simulink model "sf_car"  (R2025b)
settings: Solver=ode5  StartTime=0.0  StopTime=100  RelTol=1e-3  AbsTol=1e-6
model workspace (MAT data in the model file):
  Iei = 0.0219914882836
  converter_data = [0  137.465208994  2.232; 0.1  137.065019157  2.075; 0.2  135.864449646  1.975; 0.3  135.664354728  1.846; 0.4  137.565256453  1.72; 0.5  140.366585312  1.564; 0.6  145.268910814  1.409; 0.7  152.872517717  1.254; 0.8  162.9773111  1.096; 0.81  164.27792807  1.08; 0.82  166.178829795  1.061; 0.83  167.979684062  1.043; 0.84  170.080680706  1.028; 0.85  172.781962105  1.012; 0.86  175.383196045  1.002; 0.87  179.585189333  1.002; 0.88  183.587087703  1.001; 0.89  189.890077635  0.998; 0.9  197.693779455  0.999; 0.92  215.902417037  1.001; 0.94  244.515990379  1.002]
  downtab = [0  5  20  35; 0  5  20  35; 0  5  25  40; 0  5  30  50; 0  30  50  80; 0  30  50  80]
  downth = [0; 5; 40; 50; 90; 100]
  emap = [-40  -44  -49  -53  -57  -61  -65  -70  -74  -78  -82; 215  117  85  66  44  29  10  -2  -13  -22  -32; 245  208  178  148  122  104  85  66  48  33  18; 264  260  241  219  193  167  152  133  119  96  85; 264  279  282  275  260  238  223  208  189  171  152; 267  290  293  297  290  275  260  256  234  212  193; 267  297  305  305  305  301  293  282  267  249  226; 267  301  308  312  319  323  319  316  297  279  253; 267  301  312  319  327  327  327  327  312  293  267; 267  301  312  319  327  334  334  334  319  305  275]
  nevec = [800 1200 1600 2000 2400 2800 3200 3600 4000 4400 4800]
  p0 = 0.07934
  p1 = 0.07934
  thvec = [0; 20; 30; 40; 50; 60; 70; 80; 90; 100]
  uptab = [10  30  50  1000000; 10  30  50  1000000; 15  30  50  1000000; 23  41  60  1000000; 40  70  100  1000000; 40  70  100  1000000]
  upth = [0; 25; 35; 50; 90; 100]
  vehicledata = [3.23; 40; 0.3; 1; 50; 0]
libraries: SignalEditorBlockLib x1
settings Model: ExtModeTrigMode=oneshot  ExtModeArmWhenConnect=off  ExtModeAutoUpdateStatusClock=off  Creator=The MathWorks, Inc.  LastModifiedBy=The MathWorks, Inc.
settings SolverCC: AutoScaleAbsTol=off  AlgebraicLoopSolver=TrustRegion
settings DataIOCC: SaveFormat=Array  SaveOutput=off  SaveTime=off  ReturnWorkspaceOutputs=off  SignalLoggingName=sigsOut
settings OptimizationCC: BlockReduction=off  BooleanDataType=off  ExpressionDepthLimit=2147483647.0  InitFltsAndDblsToZero=on  EfficientMapNaN2IntZero=off  LifeSpan=inf
settings DebuggingCC: SaveWithParameterizedLinksMsg=none  UnderspecifiedInitializationDetection=Classic  MergeDetectMultiDrivingBlocksExec=none  CheckExecutionContextPreStartOutputMsg=on  SignalResolutionControl=TryResolveAllWithWarning  MultiTaskDSMMsg=warning  MultiTaskCondExecSysMsg=none  IntegerOverflowMsg=none  FcnCallInpInsideContextMsg=warning  UnconnectedInputMsg=warning  UnconnectedOutputMsg=warning  UnconnectedLineMsg=warning  StateNameClashWarn=warning  PregeneratedLibrarySubsystemCodeDiagnostic=none  SFUnexpectedBacktrackingDiag=warning  SFNoUnconditionalDefaultTransitionDiag=warning  SFExecutionAtInitializationDiag=none  IntegerSaturationMsg=none  ArithmeticOperatorsInVariantConditions=warning
settings HardwareCC: ProdBitPerPointer=32.0  ProdBitPerSizeT=32.0  ProdBitPerPtrDiffT=32.0  ProdLargestAtomicFloat=None  ProdIntDivRoundTo=Undefined  ProdEndianess=Unspecified  ProdWordSize=32.0  ProdHWDeviceType=32-bit Generic  TargetBitPerPointer=64.0  TargetBitPerSizeT=64.0  TargetBitPerPtrDiffT=64.0  TargetLongLongMode=on  TargetIntDivRoundTo=Zero  TargetEndianess=LittleEndian  TargetWordSize=64.0  TargetHWDeviceType=MATLAB Host  ProdEqTarget=off
settings ModelReferenceCC: EnableRefExpFcnMdlSchedulingChecks=on  PropagateSignalLabelsOutOfModel=off
settings SFSimCC: SFSimEcho=off  SimUseLocalCustomCode=off  SimParseCustomCode=off  CustomCodeUndefinedFunction=UseInterfaceOnly
settings RTWCC: RTWUseLocalCustomCode=off  GPUComputeCapability=3.5
settings CodeAppCC: StateflowObjectComments=on
settings GRTTargetCC: TargetFcnLib=ansi_tfl_tmw.mat  TargetLangStandard=C89/C90 (ANSI)  CombineOutputUpdateFcns=off  GRTInterface=on
settings ConfigComp: CovMetricSettings=dcmtr  CovSaveCumulativeToWorkspaceVar=on  CovSaveSingleToWorkspaceVar=on  CovExternalEMLEnable=off  CovSFcnEnable=off

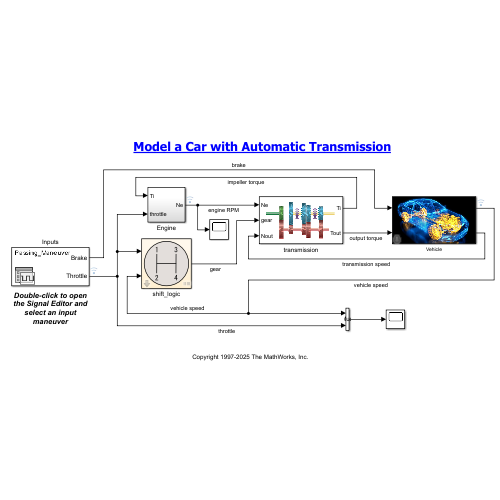
[thumbnail: Simulink's stored preview of the top-level diagram]
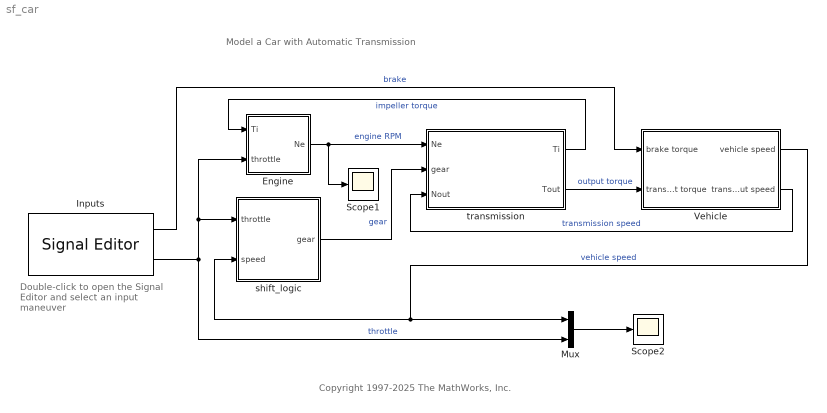
== system sf_car ==
  note: Double-click to open the Signal Editor and select an input maneuver
  note: Copyright 1997-2025 The MathWorks, Inc.
  note: Model a Car with Automatic Transmission
  Engine : Subsystem
  Inputs : SignalEditorBlockLib/Signal Editor  FileName=CarUserInput.mat  ActiveScenario=Passing_Maneuver  ActiveSignal=Throttle  IsBus=off  OutputBusObjectStr=Bus: BusObject  SampleTime=0  ZeroCross=off  OutputAfterFinalValue=Extrapolation  Unit=inherit  PreserveSignalName=on  ApplySigPropsToAllScenarios=on  ApplySigPropsToAllSignals=off  SignalPropertySource=Dialog parameters
  Mux : Mux  Inputs=2
  Scope1 : Scope
      settings: Title=Engine RPM  ActiveDisplayYMinimum=169.85512  ActiveDisplayYMaximum=4471.30392  DataLoggingSaveFormat=Array
  Scope2 : Scope
      settings: Title=Vehicle Speed & Throttle  ActiveDisplayYMinimum=-12.5  ActiveDisplayYMaximum=112.5  DataLoggingSaveFormat=Array
  Vehicle : Subsystem  mask(vehicle model){Rfd=vehicledata(1), rload0=vehicledata(2), rload2=vehicledata(3), Rw=vehicledata(4), Iv=vehicledata(5), N20=vehicledata(6)/vehicledata(4)*vehicledata(1)}
      mask prompts: Rfd "final drive ratio"; rload0 "drag friction at wheels"; rload2 "aerodynamic drag"; Rw "wheel radius"; Iv "vehicle inertia"; N20 "initial transmission output speed"
      mask help: vehicle dynamics: torque input from trans., outputs are input speed (transmission output) and vehicle speed
      mask Display: image('Henrik5000.jpg');
  shift_logic : Stateflow chart  TreatAsAtomicUnit=on  mask{TWAIT=2}
      mask prompts: TWAIT "Delay before gear change (tick)"
  transmission : Subsystem
      mask Display: image('transmission_diagram.svg')
  wires:
  transmission/1(Ti) -> Engine/1(Ti)  "impeller torque"
  Inputs/2 -> Mux/2, Engine/2(throttle), shift_logic/1(throttle)  "throttle"
  Engine/1(Ne) -> transmission/1(Ne), Scope1/1  "engine RPM"
  transmission/2(Tout) -> Vehicle/2(transmission output torque)  "output torque"
  Vehicle/2(transmission output speed) -> transmission/3(Nout)  "transmission speed"
  Vehicle/1(vehicle speed) -> Mux/1, shift_logic/2(speed)  "vehicle speed"
  Mux/1 -> Scope2/1
  Inputs/1 -> Vehicle/1(brake torque)  "brake"
  shift_logic/1(" gear") -> transmission/2(gear)  "gear"

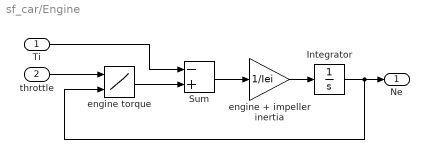
== system sf_car/Engine ==
  Ti : Inport
  throttle : Inport  Port=2
  Integrator : Integrator  InitialCondition=1000  LimitOutput=on  UpperSaturationLimit=6000  LowerSaturationLimit=600  ZeroCross=off
  Sum : Sum  Inputs=-+  InputSameDT=on  SaturateOnIntegerOverflow=on  OutDataTypeStr=Inherit: Same as first input
  engine torque : Lookup_n-D  BreakpointsForDimension1=thvec  BreakpointsForDimension2=nevec  Table=emap  InternalRulePriority=Speed
      settings: InputPortMap=u0,u1
  engine + impeller inertia : Gain  Gain=1/Iei  SaturateOnIntegerOverflow=on  OutDataTypeStr=Inherit: Same as input  ParamDataTypeStr=Inherit: Same as input
  Ne : Outport  VectorParamsAs1DForOutWhenUnconnected=off
  wires:
  Ti/1 -> Sum/1
  throttle/1 -> engine torque/1
  Integrator/1 -> engine torque/2, Ne/1
  Sum/1 -> engine + impeller inertia/1
  engine + impeller inertia/1 -> Integrator/1
  engine torque/1 -> Sum/2

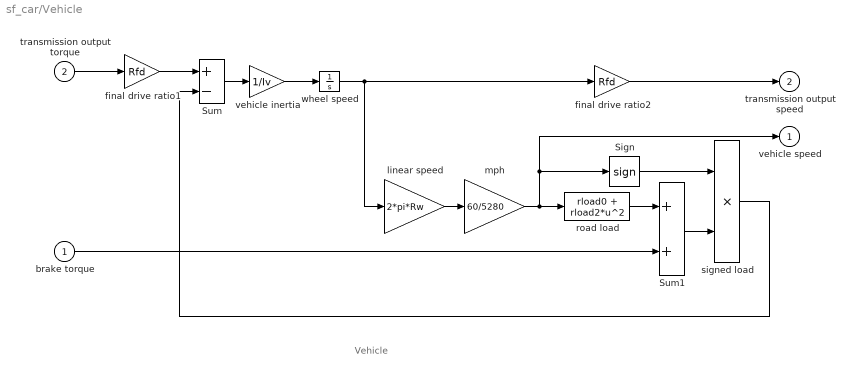
== system sf_car/Vehicle ==
  note: Vehicle
  brake torque : Inport
  transmission output torque : Inport  Port=2
  Sign : Signum
  Sum : Sum  Inputs=+-  InputSameDT=on  SaturateOnIntegerOverflow=on  OutDataTypeStr=Inherit: Same as first input
  Sum1 : Sum  InputSameDT=on  SaturateOnIntegerOverflow=on  OutDataTypeStr=Inherit: Same as first input
  final drive ratio1 : Gain  Gain=Rfd  SaturateOnIntegerOverflow=on  OutDataTypeStr=Inherit: Same as input  ParamDataTypeStr=Inherit: Same as input
  final drive ratio2 : Gain  Gain=Rfd  SaturateOnIntegerOverflow=on  OutDataTypeStr=Inherit: Same as input  ParamDataTypeStr=Inherit: Same as input
  linear speed : Gain  Gain=2*pi*Rw  SaturateOnIntegerOverflow=on  OutDataTypeStr=Inherit: Same as input  ParamDataTypeStr=Inherit: Same as input
  mph : Gain  Gain=60/5280  SaturateOnIntegerOverflow=on  OutDataTypeStr=Inherit: Same as input  ParamDataTypeStr=Inherit: Same as input
  road load : Fcn  Expr=rload0 + rload2*u^2
  signed load : Product  InputSameDT=on  SaturateOnIntegerOverflow=on  OutDataTypeStr=Inherit: Same as first input
  vehicle inertia : Gain  Gain=1/Iv  SaturateOnIntegerOverflow=on  OutDataTypeStr=Inherit: Same as input  ParamDataTypeStr=Inherit: Same as input
  wheel speed : Integrator  InitialCondition=N20/Rfd  ZeroCross=off
  vehicle speed : Outport  VectorParamsAs1DForOutWhenUnconnected=off
  transmission output speed : Outport  Port=2  VectorParamsAs1DForOutWhenUnconnected=off
  wires:
  final drive ratio2/1 -> transmission output speed/1
  brake torque/1 -> Sum1/2
  Sum1/1 -> signed load/2
  road load/1 -> Sum1/1
  Sign/1 -> signed load/1
  signed load/1 -> Sum/2
  transmission output torque/1 -> final drive ratio1/1
  vehicle inertia/1 -> wheel speed/1
  Sum/1 -> vehicle inertia/1
  mph/1 -> vehicle speed/1, Sign/1, road load/1
  linear speed/1 -> mph/1
  wheel speed/1 -> linear speed/1, final drive ratio2/1
  final drive ratio1/1 -> Sum/1

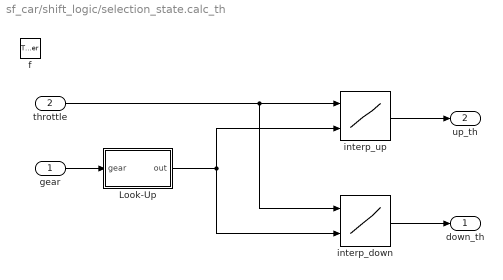
== system sf_car/shift_logic/selection_state.calc_th ==
  gear : Inport  OutDataTypeStr=Enum: gearType  PortDimensions=1
  throttle : Inport  Port=2  OutDataTypeStr=double  PortDimensions=1
  f : TriggerPort  TriggerType=function-call  VariantControl=Variant
      settings: CopyFcn=Stateflow.SLINSF.SimulinkMan.removeBlockPreDeleteFcn  PreDeleteFcn=Stateflow.SLINSF.SimulinkMan.unsafePredeleteFcn
  Look-Up : MATLAB Function  TreatAsAtomicUnit=on
  interp_down : Lookup_n-D  BreakpointsForDimension1=downth  BreakpointsForDimension2=[1:4]  Table=downtab
      settings: InputPortMap=u0,u1
  interp_up : Lookup_n-D  BreakpointsForDimension1=upth  BreakpointsForDimension2=[1:4]  Table=uptab
      settings: InputPortMap=u0,u1
  down_th : Outport  VectorParamsAs1DForOutWhenUnconnected=off
  up_th : Outport  Port=2  VectorParamsAs1DForOutWhenUnconnected=off
  wires:
  interp_up/1 -> up_th/1
  interp_down/1 -> down_th/1
  throttle/1 -> interp_down/1, interp_up/1
  gear/1 -> Look-Up/1(gear)
  Look-Up/1(out) -> interp_down/2, interp_up/2

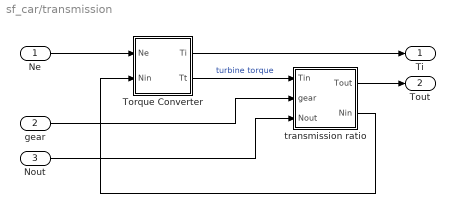
== system sf_car/transmission ==
  Ne : Inport
  gear : Inport  Port=2
  Nout : Inport  Port=3
  Torque Converter : Subsystem  mask(torque converter){speedratio=converter_data(:,1), Kfactor=converter_data(:,2), Torkratio=converter_data(:,3)}
      mask prompts: speedratio "speed ratio"; Kfactor "K factor"; Torkratio "torque ratio"
      mask help: torque converter
      mask Help: Torque converter input and output torques are computed as a function of the input and output speeds
      mask Display: plot([cos([90:10:450]*pi/180),.63*cos([90:10:450]*pi/180),.63*cos([90:10:240]*pi/180),cos([240:10:300]*pi/180),.63*cos([300]*pi/180)],[sin([90:10:450]*pi/180),.63*sin([90:10:450]*pi/180)+.1,.63*sin([90:10:240]*pi/180)+.1,sin([240:10:300]*pi/180),.63*sin([300]*pi/180)+.1])
  transmission ratio : Subsystem
  Ti : Outport  VectorParamsAs1DForOutWhenUnconnected=off
  Tout : Outport  Port=2  VectorParamsAs1DForOutWhenUnconnected=off
  wires:
  transmission ratio/1(Tout) -> Tout/1
  Torque Converter/1(Ti) -> Ti/1
  Nout/1 -> transmission ratio/3(Nout)
  gear/1 -> transmission ratio/2(gear)
  Ne/1 -> Torque Converter/1(Ne)
  transmission ratio/2(Nin) -> Torque Converter/2(Nin)
  Torque Converter/2(Tt) -> transmission ratio/1(Tin)  "turbine torque"

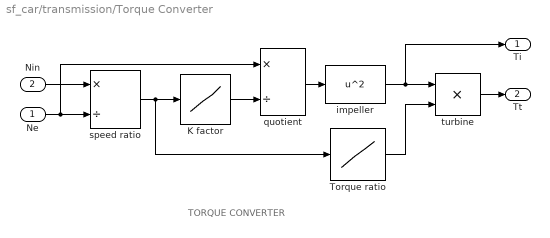
== system sf_car/transmission/Torque Converter ==
  note: TORQUE CONVERTER
  Ne : Inport
  Nin : Inport  Port=2
  K factor : Lookup_n-D  NumberOfTableDimensions=1  BreakpointsForDimension1=speedratio  Table=Kfactor  InternalRulePriority=Speed  SaturateOnIntegerOverflow=on
  Torque ratio : Lookup_n-D  NumberOfTableDimensions=1  BreakpointsForDimension1=speedratio  Table=Torkratio  InternalRulePriority=Speed  SaturateOnIntegerOverflow=on
  impeller : Fcn  Expr=u^2
  quotient : Product  Inputs=*/  InputSameDT=on  SaturateOnIntegerOverflow=on  OutDataTypeStr=Inherit: Same as first input
  speed ratio : Product  Inputs=*/  InputSameDT=on  SaturateOnIntegerOverflow=on  OutDataTypeStr=Inherit: Same as first input
  turbine : Product  InputSameDT=on  SaturateOnIntegerOverflow=on  OutDataTypeStr=Inherit: Same as first input
  Ti : Outport  VectorParamsAs1DForOutWhenUnconnected=off
  Tt : Outport  Port=2  VectorParamsAs1DForOutWhenUnconnected=off
  wires:
  Torque ratio/1 -> turbine/2
  quotient/1 -> impeller/1
  K factor/1 -> quotient/2
  speed ratio/1 -> Torque ratio/1, K factor/1
  impeller/1 -> turbine/1, Ti/1
  turbine/1 -> Tt/1
  Ne/1 -> speed ratio/2, quotient/1
  Nin/1 -> speed ratio/1

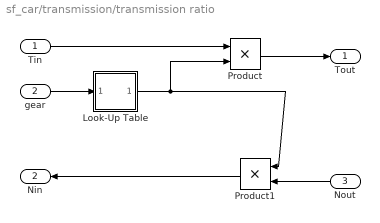
== system sf_car/transmission/transmission ratio ==
  Tin : Inport
  gear : Inport  Port=2
  Nout : Inport  Port=3
  Look-Up Table : MATLAB Function  TreatAsAtomicUnit=on
  Product : Product  InputSameDT=on  SaturateOnIntegerOverflow=on  OutDataTypeStr=Inherit: Same as first input
  Product1 : Product  InputSameDT=on  SaturateOnIntegerOverflow=on  OutDataTypeStr=Inherit: Same as first input
  Tout : Outport  VectorParamsAs1DForOutWhenUnconnected=off
  Nin : Outport  Port=2  VectorParamsAs1DForOutWhenUnconnected=off
  wires:
  Look-Up Table/1(out) -> Product1/1, Product/2
  Nout/1 -> Product1/2
  Product1/1 -> Nin/1
  Product/1 -> Tout/1
  Tin/1 -> Product/1
  gear/1 -> Look-Up Table/1(gear)

== stateflow chart sf_car/shift_logic ==
  settings: updateMethod=DISCRETE  sampleTime=0.04
  state gear_state [parallel]
    settings: executionOrder=1
    state first
    state second
    state third
    state fourth
    (default) -> first
    second -> third [order 1] : UP
    third -> fourth [order 1] : UP
    first -> second : UP
    fourth -> third : DOWN
    third -> second [order 2] : DOWN
    second -> first [order 2] : DOWN
  state selection_state [parallel]
    during: [down_th,up_th] = calc_th(gear,throttle);
    settings: executionOrder=2
    state steady_state
    state downshifting
    state upshifting
    state [down_th,up_th] = calc_th(gear,throttle) [function]
    (default) -> steady_state
    steady_state -> upshifting [order 1] : [speed > up_th]
    steady_state -> downshifting [order 2] : [speed < down_th]
    downshifting -> steady_state [order 1] : after(TWAIT,tick)
        | [speed <= down_th]
        | {send(gear_state.DOWN)}
    downshifting -> steady_state [order 2] : [speed > down_th]
    upshifting -> steady_state [order 1] : after(TWAIT,tick)
        | [speed >= up_th]
        | {send(gear_state.UP)}
    upshifting -> steady_state [order 2] : [speed < up_th]
  data: gear function_input Enum: gearType size=1; throttle function_input double size=1; down_th function_output; up_th function_output; TWAIT parameter uint8; up_th local double; down_th local double; throttle input; speed input double; gear output Enum: gearType
  events: DOWN local EITHER_EDGE_EVENT; UP local EITHER_EDGE_EVENT

== matlab function sf_car/transmission/transmission ratio/Look-Up Table ==
  data: gear input; out output
function out = fcn(gear)
    %#codegen
    table = [2.393 1.450 1.000 0.677];
    switch(gear)
        case gearType.fourth
            out=table(4);        
        case gearType.third
            out=table(3);            
        case gearType.second
            out=table(2);
        otherwise % gearType.first
            out=table(1);
    end
    
end

== matlab function sf_car/shift_logic/selection_state.calc_th/Look-Up ==
  data: gear input; out output
function out = fcn(gear)
    %#codegen
    table = [1 2 3 4];
    switch(gear)
        case gearType.fourth;
            out=table(4);        
        case gearType.third;
            out=table(3);
        case gearType.second;
            out=table(2);            
        otherwise; % gearType.first
            out=table(1);
    end
    
end
